simulink model "Two_stage_NIBB"  (R2022a)
settings: Solver=VariableStepAuto  StartTime=0.0  StopTime=0.5  RelTol=1e-3
libraries: spsSeriesRLCBranchLib x8, spsDiodeLib x6, spsMosfetLib x6, spsVoltageMeasurementLib x3, spsCurrentMeasurementLib x2, eePowerMeasurement x2, spsDCVoltageSourceLib x1, spsMeanLib x1, spspowerguiLib x1
settings Model: Creator=Bobby  LastModifiedBy=Bobby

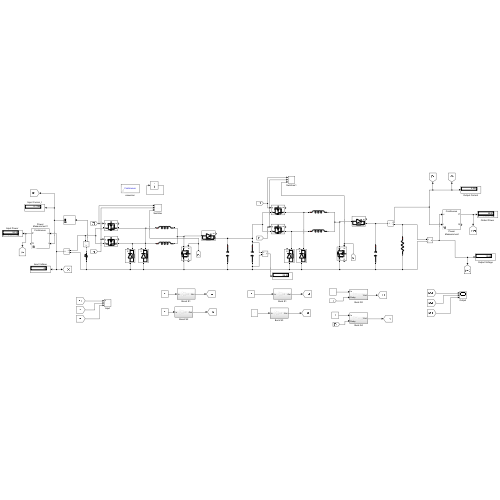
[thumbnail: Simulink's stored preview of the top-level diagram]
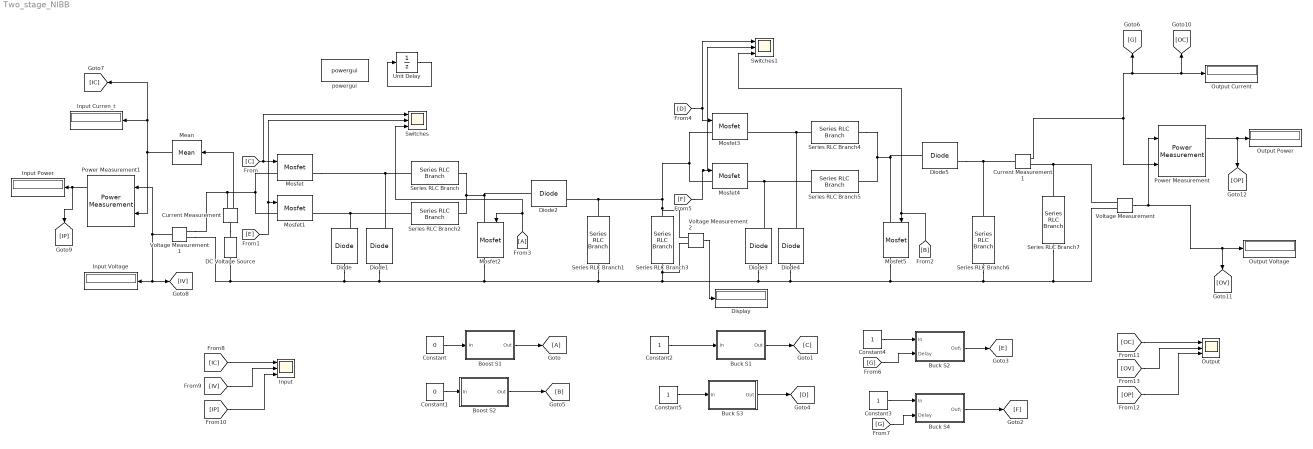
== system Two_stage_NIBB ==
  Boost S1 : Subsystem
  Boost S2 : Subsystem
  Buck S1 : Subsystem
  Buck S2 : Subsystem
  Buck S3 : Subsystem
  Buck S4 : Subsystem
  Constant : Constant  Value=0
  Constant1 : Constant  Value=0
  Constant{2..5} (4 alike) : Constant
  Current Measurement : spsCurrentMeasurementLib/Current Measurement  PhasorSimulation=off  OutputType=Complex  PSBequivalent=0
  Current Measurement1 : spsCurrentMeasurementLib/Current Measurement  PhasorSimulation=off  OutputType=Complex  PSBequivalent=0
  DC Voltage Source : spsDCVoltageSourceLib/DC Voltage Source  Amplitude=48  Measurements=None
  Diode{,1..5} (6 alike) : spsDiodeLib/Diode  Ron=0.001  Lon=0  Vf=0.8  IC=0  UseSnubber=0  Rs=500  Cs=250e-9  Measurements=on
  Display : Display
  From3 : From
  Goto : Goto
  Input : Scope  NumInputPorts=3
  Input Curren_t : Display
  Input Power : Display
  Input Voltage : Display
  Mean : spsMeanLib/Mean  Freq=60  Vinit=0  Ts=0
  Mosfet{,1..5} (6 alike) : spsMosfetLib/Mosfet  Ron=0.1  Lon=0  Rd=0.01  Vfd=0  IC=0  Rs=1e5  Cs=inf  Measurements=on
  Output : Scope  NumInputPorts=3
  Output Current : Display
  Output Power : Display
  Output Voltage : Display
  Power Measurement : eePowerMeasurement/Power Measurement  LabelModeActiveChoice=Continuous  F=60  K=[0 1 2 3]  Ts=0
      settings: SourceProductBaseCode=PS
  Power Measurement1 : eePowerMeasurement/Power Measurement  LabelModeActiveChoice=Continuous  F=60  K=[0 1 2 3]  Ts=0
      settings: SourceProductBaseCode=PS
  Series RLC Branch{,2,4..5} (4 alike) : spsSeriesRLCBranchLib/Series RLC Branch  LConnTagsString=__new0  RConnTagsString=__new0  BranchType=L  Resistance=1  Inductance=80e-6  SetiL0=off  InitialCurrent=0  Capacitance=1e-6  Setx0=off  InitialVoltage=0  Measurements=None
  Series RLC Branch1 : spsSeriesRLCBranchLib/Series RLC Branch  LConnTagsString=__new0  RConnTagsString=__new0  BranchType=C  Resistance=1  Inductance=1e-3  SetiL0=off  InitialCurrent=0  Capacitance=1666e-6  Setx0=off  InitialVoltage=0  Measurements=None
  Series RLC Branch3 : spsSeriesRLCBranchLib/Series RLC Branch  LConnTagsString=__new0  RConnTagsString=__new0  BranchType=C  Resistance=1  Inductance=1e-3  SetiL0=off  InitialCurrent=0  Capacitance=450e-6  Setx0=off  InitialVoltage=0  Measurements=None
  Series RLC Branch6 : spsSeriesRLCBranchLib/Series RLC Branch  LConnTagsString=__new0  RConnTagsString=__new0  BranchType=C  Resistance=1  Inductance=1e-3  SetiL0=off  InitialCurrent=0  Capacitance=1666e-6  Setx0=off  InitialVoltage=0  Measurements=None
  Series RLC Branch7 : spsSeriesRLCBranchLib/Series RLC Branch  LConnTagsString=__new0  RConnTagsString=__new0  BranchType=R  Resistance=5.76  Inductance=1e-3  SetiL0=off  InitialCurrent=0  Capacitance=1e-6  Setx0=off  InitialVoltage=0  Measurements=None
  Switches : Scope  NumInputPorts=3
  Switches1 : Scope  NumInputPorts=3
  Unit Delay : UnitDelay  SampleTime=-1  HasFrameUpgradeWarning=on
  Voltage Measurement : spsVoltageMeasurementLib/Voltage Measurement  PhasorSimulation=off  OutputType=Complex  PSBequivalent=0
  Voltage Measurement1 : spsVoltageMeasurementLib/Voltage Measurement  PhasorSimulation=off  OutputType=Complex  PSBequivalent=0
  Voltage Measurement2 : spsVoltageMeasurementLib/Voltage Measurement  PhasorSimulation=off  OutputType=Complex  PSBequivalent=0
  powergui : spspowerguiLib/powergui  Priority=1  SimulationMode=Continuous  SampleTime=50e-6  frequency=60  Iterations=50  frequencyindice=0  Pbase=100e6  ErrMax=1e-4  UnitsV=kV  UnitsW=MW  buscounter=0  FunctionMessages=off  echomessages=off  EnableUseOfTLC=off  CurrentSourceSwitches=off  DisableSnubberDevices=off  DisableRonSwitches=off  DisableVfSwitches=off  DisplayEquations=off  AutomaticDiscreteSolvers=off  SolverType=Tustin/Backward Euler (TBE)  Interpol=off  ExternalGateDelay=off  methode=off  Ts=100  x0status=blocks  SPID=on  SwTol=0  HookPort=off  NonlinearTolerance=1e-4  nMaxIteration=100  ContinueOnMaxIteration=off  RestoreLinks=warning  ResistiveCurrentMeasurement=off  Frange=[0:2:500]  Ylog=off  Xlog=on  ShowGrid=off  save=off  variable=ZData  structure=0  ZoomFFT=off  StartTime=0.0  cycles=1  DisplayStyle=1  fundamental=60  FreqAxis=off  MaxFrequency=1000  frequencyindicesteady=1  RmsSteady=1  display=off
  wires:
  Voltage Measurement1/1 -> [IV], Input Voltage/1, Power Measurement1/1
  Power Measurement1/1 -> [IP], Input Power/1
  Voltage Measurement/1 -> [OV], Output Voltage/1, Power Measurement/1
  Current Measurement1/1 -> Power Measurement/2, Output Current/1, [OC], [G]
  Power Measurement/1 -> [OP], Output Power/1
  Unit Delay/1 -> Unit Delay/1
  Boost S1/1(Out) -> Goto/1
  Boost S2/1(Out) -> [B]
  Buck S1/1(Out) -> [C]
  Buck S3/1(Out) -> [D]
  Buck S2/1(Out\) -> [E]
  Buck S4/1(Out\) -> [F]
  Constant/1 -> Boost S1/1(In)
  Constant1/1 -> Boost S2/1(In)
  Constant2/1 -> Buck S1/1(In)
  Constant5/1 -> Buck S3/1(In)
  Constant4/1 -> Buck S2/1(In)
  Constant3/1 -> Buck S4/1(In)
  [C] -> Switches/1, Mosfet/1
  [E] -> Switches/2, Mosfet1/1
  From3/1 -> Switches/3, Mosfet2/1
  [B] -> Switches1/3, Mosfet5/1
  [D] -> Switches1/1, Mosfet3/1
  [F] -> Switches1/2, Mosfet4/1
  [G] -> Buck S2/2(Delay)
  [G] -> Buck S4/2(Delay)
  Voltage Measurement2/1 -> Display/1
  [IC] -> Input/1
  [IV] -> Input/2
  [IP] -> Input/3
  [OC] -> Output/1
  [OP] -> Output/3
  [OV] -> Output/2
  Current Measurement/1 -> Mean/1
  Mean/1 -> Power Measurement1/2, Input Curren_t/1, [IC]
  connections:
  Mosfet/RConn1 -- Diode1/RConn1 -- Series RLC Branch/LConn1
  Series RLC Branch2/LConn1 -- Mosfet1/RConn1 -- Diode/RConn1
  Mosfet1/LConn1 -- Current Measurement/RConn1 -- Voltage Measurement1/LConn1 -- Mosfet/LConn1
  Diode/LConn1 -- Series RLC Branch1/RConn1 -- Voltage Measurement2/LConn2 -- Series RLC Branch3/RConn1 -- Voltage Measurement/LConn2 -- Series RLC Branch7/RConn1 -- Series RLC Branch6/RConn1 -- Mosfet5/RConn1 -- Diode4/LConn1 -- Diode3/LConn1 -- Mosfet2/RConn1 -- Diode1/LConn1 -- Voltage Measurement1/LConn2 -- DC Voltage Source/LConn1
  Series RLC Branch/RConn1 -- Series RLC Branch2/RConn1 -- Mosfet2/LConn1 -- Diode2/LConn1
  Series RLC Branch1/LConn1 -- Voltage Measurement2/LConn1 -- Series RLC Branch3/LConn1 -- Mosfet3/LConn1 -- Mosfet4/LConn1 -- Diode2/RConn1
  Series RLC Branch4/LConn1 -- Mosfet3/RConn1 -- Diode4/RConn1
  Series RLC Branch5/LConn1 -- Mosfet4/RConn1 -- Diode3/RConn1
  Series RLC Branch4/RConn1 -- Mosfet5/LConn1 -- Diode5/LConn1 -- Series RLC Branch5/RConn1
  Diode5/RConn1 -- Current Measurement1/LConn1 -- Series RLC Branch6/LConn1
  Series RLC Branch7/LConn1 -- Voltage Measurement/LConn1 -- Current Measurement1/RConn1
  Current Measurement/LConn1 -- DC Voltage Source/RConn1

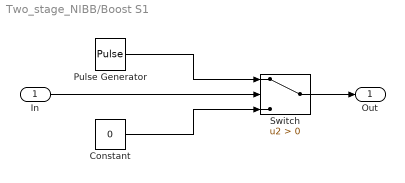
== system Two_stage_NIBB/Boost S1 ==
  In : Inport
  Constant : Constant  Value=0
  Pulse Generator : DiscretePulseGenerator  PulseType=Time based  Period=20e-6  PulseWidth=52.5
  Switch : Switch  Criteria=u2 > Threshold  SaturateOnIntegerOverflow=off  InputSameDT=off
  Out : Outport
  wires:
  Pulse Generator/1 -> Switch/1
  Constant/1 -> Switch/3
  In/1 -> Switch/2
  Switch/1 -> Out/1

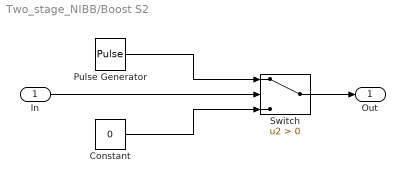
== system Two_stage_NIBB/Boost S2 ==
  In : Inport
  Constant : Constant  Value=0
  Pulse Generator : DiscretePulseGenerator  PulseType=Time based  Period=20e-6  PulseWidth=52.5
  Switch : Switch  Criteria=u2 > Threshold  SaturateOnIntegerOverflow=off  InputSameDT=off
  Out : Outport
  wires:
  Pulse Generator/1 -> Switch/1
  Constant/1 -> Switch/3
  In/1 -> Switch/2
  Switch/1 -> Out/1

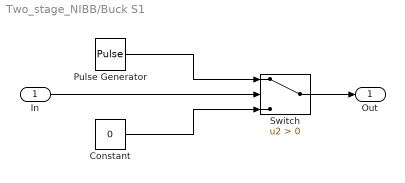
== system Two_stage_NIBB/Buck S1 ==
  In : Inport
  Constant : Constant  Value=0
  Pulse Generator : DiscretePulseGenerator  PulseType=Time based  Period=20e-6  PulseWidth=52.5
  Switch : Switch  Criteria=u2 > Threshold  SaturateOnIntegerOverflow=off  InputSameDT=off
  Out : Outport
  wires:
  Pulse Generator/1 -> Switch/1
  Constant/1 -> Switch/3
  In/1 -> Switch/2
  Switch/1 -> Out/1

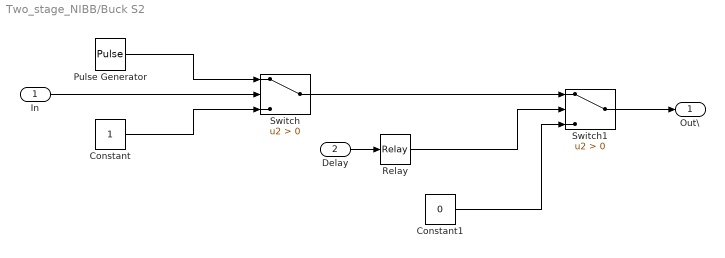
== system Two_stage_NIBB/Buck S2 ==
  In : Inport
  Delay : Inport  Port=2
  Constant : Constant
  Constant1 : Constant  Value=0
  Pulse Generator : DiscretePulseGenerator  PulseType=Time based  Period=20e-6  PulseWidth=52.5  PhaseDelay=10e-6
  Relay : Relay  OnSwitchValue=11  OffSwitchValue=10.8
  Switch : Switch  Criteria=u2 > Threshold  SaturateOnIntegerOverflow=off  InputSameDT=off
  Switch1 : Switch  Criteria=u2 > Threshold  SaturateOnIntegerOverflow=off  InputSameDT=off
  Out\ : Outport
  wires:
  Pulse Generator/1 -> Switch/1
  Constant/1 -> Switch/3
  In/1 -> Switch/2
  Switch/1 -> Switch1/1
  Relay/1 -> Switch1/2
  Delay/1 -> Relay/1
  Constant1/1 -> Switch1/3
  Switch1/1 -> Out\/1

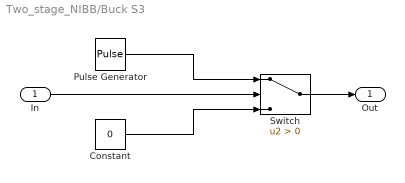
== system Two_stage_NIBB/Buck S3 ==
  In : Inport
  Constant : Constant  Value=0
  Pulse Generator : DiscretePulseGenerator  PulseType=Time based  Period=20e-6  PulseWidth=52.5
  Switch : Switch  Criteria=u2 > Threshold  SaturateOnIntegerOverflow=off  InputSameDT=off
  Out : Outport
  wires:
  Pulse Generator/1 -> Switch/1
  Constant/1 -> Switch/3
  In/1 -> Switch/2
  Switch/1 -> Out/1

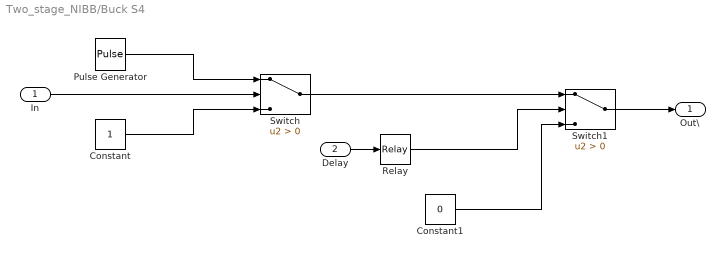
== system Two_stage_NIBB/Buck S4 ==
  In : Inport
  Delay : Inport  Port=2
  Constant : Constant
  Constant1 : Constant  Value=0
  Pulse Generator : DiscretePulseGenerator  PulseType=Time based  Period=20e-6  PulseWidth=55  PhaseDelay=10e-6
  Relay : Relay  OnSwitchValue=11  OffSwitchValue=10.8
  Switch : Switch  Criteria=u2 > Threshold  SaturateOnIntegerOverflow=off  InputSameDT=off
  Switch1 : Switch  Criteria=u2 > Threshold  SaturateOnIntegerOverflow=off  InputSameDT=off
  Out\ : Outport
  wires:
  Pulse Generator/1 -> Switch/1
  Constant/1 -> Switch/3
  In/1 -> Switch/2
  Switch/1 -> Switch1/1
  Relay/1 -> Switch1/2
  Delay/1 -> Relay/1
  Constant1/1 -> Switch1/3
  Switch1/1 -> Out\/1
